simulink model "s_b4a4x256f"  (R2016b)
settings: Solver=VariableStepDiscrete  StartTime=0.0  StopTime=1  RelTol=1e-3
undefined symbols (not defined in the file): fft_stages, n_bits_ants, n_bits_xengs
libraries: xbsIndex_r4 x19303, casper_library_misc x166, casper_library_scopes x10, xbsReplacements_r4 x9, casper_library_delays x8, xps_library x3
(part 47 of 165)

== system s_b4a4x256f/sys0/31->32/conv8 ==
  note: (ones_bit & 1) -> round-to-even
      | (ones_bit ^ 1) -> round-to-odd
      | (sign_bit & 1)-> round-to-zero
      | (sign_bit ^ 1) -> round-to-inf
      | (X ~| 1) -> round half down
      | (X | 1) -> round half up
  in : Inport
  Concat : xbsIndex_r4/Concat  num_inputs=2  dbl_ovrd=off  block_type=concat
      settings: block_version=10.1.3
  Constant : xbsIndex_r4/Constant  const=1  gui_display_data_type=Fixed-point  arith_type=Unsigned  n_bits=1  bin_pt=0  preci_type=Single  exp_width=8  frac_width=24  explicit_period=off  period=1  equ=P=C  opselect=C  inp2=PCIN>>17  opr=+  inp1=P  carry=CIN  dbl_ovrd=off  block_type=constant
  Reinterpret : xbsIndex_r4/Reinterpret  force_arith_type=on  arith_type=Unsigned  force_bin_pt=on  bin_pt=0  block_type=reinterpret
      settings: infoedit="Changes signal type without altering the binary representation.   You can changed the signal between signed and unsigned, and relocate the binary point.<P><P>Hardware notes: In hardware this block costs nothing.<P><P>Example:  Suppose the input is 6 bits wide, signed, with 2 fractional bits, and the output is forced to unsigned with 0 fractional bits.  Then an input of -2.0 (1110.00 in binary 2's complement) becomes an output of 56 (111000 in binary)."  block_version=10.1.3
  adder : xbsIndex_r4/AddSub  mode=Addition  use_carryin=off  use_carryout=off  en=off  latency=0  precision=User Defined  arith_type="Signed  (2's comp)"  n_bits=32  bin_pt=0  quantization=Truncate  overflow=Wrap  use_behavioral_HDL=off  hw_selection=Fabric  pipelined=on  use_rpm=on  dbl_ovrd=off  block_type=addsub
      settings: xl_area=[0, 0, 0, 0, 0, 0, 0]  block_version=10.1.3
  almost_half : xbsIndex_r4/Constant  const=0  gui_display_data_type=Fixed-point  arith_type=Unsigned  n_bits=1  bin_pt=0  preci_type=Single  exp_width=8  frac_width=24  explicit_period=off  period=1  equ=P=C  opselect=C  inp2=PCIN>>17  opr=+  inp1=P  carry=CIN  dbl_ovrd=off  block_type=constant
  bit : xbsIndex_r4/Slice  nbits=1  boolean_output=off  mode=Lower Bit Location + Width  bit1=0  base1=MSB of Input  bit0=0  base0=LSB of Input  dbl_ovrd=off  block_type=slice
      settings: infoedit="Extracts a given range of bits from each input sample and presents it at the output.  The output type is ordinarily unsigned with binary point at zero, but can be Boolean when the slice is one bit wide.<P><P>Hardware notes: In hardware this block costs nothing."  block_version=10.1.3
  force1 : xbsIndex_r4/Reinterpret  force_arith_type=on  arith_type="Signed  (2's comp)"  force_bin_pt=on  bin_pt=1  block_type=reinterpret
      settings: infoedit="Changes signal type without altering the binary representation.   You can changed the signal between signed and unsigned, and relocate the binary point.<P><P>Hardware notes: In hardware this block costs nothing.<P><P>Example:  Suppose the input is 6 bits wide, signed, with 2 fractional bits, and the output is forced to unsigned with 0 fractional bits.  Then an input of -2.0 (1110.00 in binary 2's complement) becomes an output of 56 (111000 in binary)."  block_version=10.1.3
  force2 : xbsIndex_r4/Reinterpret  force_arith_type=off  arith_type="Signed  (2's comp)"  force_bin_pt=on  bin_pt=1  block_type=reinterpret
      settings: infoedit="Changes signal type without altering the binary representation.   You can changed the signal between signed and unsigned, and relocate the binary point.<P><P>Hardware notes: In hardware this block costs nothing.<P><P>Example:  Suppose the input is 6 bits wide, signed, with 2 fractional bits, and the output is forced to unsigned with 0 fractional bits.  Then an input of -2.0 (1110.00 in binary 2's complement) becomes an output of 56 (111000 in binary)."  block_version=10.1.3
  tweak_op : xbsIndex_r4/Logical  logical_function=NOR  inputs=2  en=off  latency=0  precision=Full  arith_type=Unsigned  n_bits=8  bin_pt=2  align_bp=on  dbl_ovrd=off  block_type=logical
      settings: xl_area=[0, 0, 0, 0, 0, 0, 0]
  out : Outport
  wires:
  tweak_op/1 -> Concat/2
  Constant/1 -> tweak_op/2
  bit/1 -> tweak_op/1
  almost_half/1 -> force2/1
  in/1 -> Reinterpret/1, bit/1
  Concat/1 -> force1/1
  Reinterpret/1 -> Concat/1
  force1/1 -> adder/1
  force2/1 -> adder/2
  adder/1 -> out/1

== system s_b4a4x256f/sys0/31->32/debus ==
  bus_in : Inport
  reinterpret{1..8} (8 alike) : xbsIndex_r4/Reinterpret  force_arith_type=on  arith_type="Signed  (2's comp)"  force_bin_pt=on  bin_pt=0  block_type=reinterpret
  slice1 : xbsIndex_r4/Slice  nbits=31  boolean_output=off  mode=Upper Bit Location + Width  bit1=-217  base1=MSB of Input  bit0=0  base0=LSB of Input  dbl_ovrd=off  block_type=slice
  slice2 : xbsIndex_r4/Slice  nbits=31  boolean_output=off  mode=Upper Bit Location + Width  bit1=-186  base1=MSB of Input  bit0=0  base0=LSB of Input  dbl_ovrd=off  block_type=slice
  slice3 : xbsIndex_r4/Slice  nbits=31  boolean_output=off  mode=Upper Bit Location + Width  bit1=-155  base1=MSB of Input  bit0=0  base0=LSB of Input  dbl_ovrd=off  block_type=slice
  slice4 : xbsIndex_r4/Slice  nbits=31  boolean_output=off  mode=Upper Bit Location + Width  bit1=-124  base1=MSB of Input  bit0=0  base0=LSB of Input  dbl_ovrd=off  block_type=slice
  slice5 : xbsIndex_r4/Slice  nbits=31  boolean_output=off  mode=Upper Bit Location + Width  bit1=-93  base1=MSB of Input  bit0=0  base0=LSB of Input  dbl_ovrd=off  block_type=slice
  slice6 : xbsIndex_r4/Slice  nbits=31  boolean_output=off  mode=Upper Bit Location + Width  bit1=-62  base1=MSB of Input  bit0=0  base0=LSB of Input  dbl_ovrd=off  block_type=slice
  slice7 : xbsIndex_r4/Slice  nbits=31  boolean_output=off  mode=Upper Bit Location + Width  bit1=-31  base1=MSB of Input  bit0=0  base0=LSB of Input  dbl_ovrd=off  block_type=slice
  slice8 : xbsIndex_r4/Slice  nbits=31  boolean_output=off  mode=Upper Bit Location + Width  bit1=0  base1=MSB of Input  bit0=0  base0=LSB of Input  dbl_ovrd=off  block_type=slice
  msb_out8 : Outport
  out7 : Outport  Port=2
  out6 : Outport  Port=3
  out5 : Outport  Port=4
  out4 : Outport  Port=5
  out3 : Outport  Port=6
  out2 : Outport  Port=7
  lsb_out1 : Outport  Port=8
  wires:
  bus_in/1 -> slice8/1, slice7/1, slice6/1, slice5/1, slice4/1, slice3/1, slice2/1, slice1/1
  slice8/1 -> reinterpret8/1
  reinterpret8/1 -> msb_out8/1
  slice7/1 -> reinterpret7/1
  reinterpret7/1 -> out7/1
  slice6/1 -> reinterpret6/1
  reinterpret6/1 -> out6/1
  slice5/1 -> reinterpret5/1
  reinterpret5/1 -> out5/1
  slice4/1 -> reinterpret4/1
  reinterpret4/1 -> out4/1
  slice3/1 -> reinterpret3/1
  reinterpret3/1 -> out3/1
  slice2/1 -> reinterpret2/1
  reinterpret2/1 -> out2/1
  slice1/1 -> reinterpret1/1
  reinterpret1/1 -> lsb_out1/1

== system s_b4a4x256f/sys0/beng_tvg/Delay10 ==
  d : Inport
  q : Outport
  wires:
  d/1 -> q/1

== system s_b4a4x256f/sys0/beng_tvg/Delay11 ==
  d : Inport
  q : Outport
  wires:
  d/1 -> q/1

== system s_b4a4x256f/sys0/beng_tvg/Delay52 ==
  d : Inport
  Register0 : xbsIndex_r4/Register  init=0  rst=off  en=off  dbl_ovrd=off  block_type=register
      settings: block_version=11.4
  q : Outport
  wires:
  Register0/1 -> q/1
  d/1 -> Register0/1

== system s_b4a4x256f/sys0/beng_tvg/Delay9 ==
  d : Inport
  q : Outport
  wires:
  d/1 -> q/1

== system s_b4a4x256f/sys0/bf/fbf ==
  note: beam filtering
  note: requanitse
  note: accumulate
  note: combine data from different antennas into beams
  note: beam steering
  note: antenna beam weights
  note: split polarisations and
      | duplicate for multiple beams
  note: TODO
  note: control interface
  note: TODO
  di : Inport
  deni : Inport  Port=2
  badi : Inport  Port=3
  timei : Inport  Port=4
  misci : Inport  Port=5
  ld_antenna : Inport  Port=6
  ld_stream : Inport  Port=7
  Assert1 : xbsIndex_r4/Assert  assert_type=on  type_source=Explicitly  gui_display_data_type=Boolean  arith_type=Boolean  n_bits=16  bin_pt=14  preci_type=Single  exp_width=8  frac_width=24  assert_rate=off  rate_source=Explicitly  period=1  output_port=on  block_type=assert
  Assert2 : xbsIndex_r4/Assert  assert_type=on  type_source=Explicitly  gui_display_data_type=Boolean  arith_type=Boolean  n_bits=16  bin_pt=14  preci_type=Single  exp_width=8  frac_width=24  assert_rate=off  rate_source=Explicitly  period=1  output_port=on  block_type=assert
  Assert3 : xbsIndex_r4/Assert  assert_type=on  type_source=Explicitly  gui_display_data_type=Fixed-point  arith_type=Unsigned  n_bits=n_bits_in*2*2^polarisation_bits  bin_pt=0  preci_type=Single  exp_width=8  frac_width=24  assert_rate=off  rate_source=Explicitly  period=1  output_port=on  block_type=assert
  Assert4 : xbsIndex_r4/Assert  assert_type=on  type_source=Explicitly  gui_display_data_type=Fixed-point  arith_type=Unsigned  n_bits=timestamp_bits  bin_pt=0  preci_type=Single  exp_width=8  frac_width=24  assert_rate=off  rate_source=Explicitly  period=1  output_port=on  block_type=assert
  Assert6 : xbsIndex_r4/Assert  assert_type=on  type_source=Explicitly  gui_display_data_type=Fixed-point  arith_type=Unsigned  n_bits=ant_bits  bin_pt=0  preci_type=Single  exp_width=8  frac_width=24  assert_rate=off  rate_source=Explicitly  period=1  output_port=on  block_type=assert
  Assert7 : xbsIndex_r4/Assert  assert_type=on  type_source=Explicitly  gui_display_data_type=Fixed-point  arith_type=Unsigned  n_bits=polarisation_bits+beam_bits  bin_pt=0  preci_type=Single  exp_width=8  frac_width=24  assert_rate=off  rate_source=Explicitly  period=1  output_port=on  block_type=assert
  Concat : xbsIndex_r4/Concat  num_inputs=2  dbl_ovrd=off  block_type=concat
  Concat1 : xbsIndex_r4/Concat  num_inputs=3  dbl_ovrd=off  block_type=concat
  Concat2 : xbsIndex_r4/Concat  num_inputs=2  dbl_ovrd=off  block_type=concat
  Concat3 : xbsIndex_r4/Concat  num_inputs=2  dbl_ovrd=off  block_type=concat
  Constant : xbsIndex_r4/Constant  const=0  gui_display_data_type=Boolean  arith_type=Boolean  n_bits=16  bin_pt=14  preci_type=Single  exp_width=8  frac_width=24  explicit_period=on  period=1  equ=P=C  opselect=C  inp2=PCIN>>17  opr=+  inp1=P  carry=CIN  dbl_ovrd=off  block_type=constant
  Constant1 : xbsIndex_r4/Constant  const=0  gui_display_data_type=Fixed-point  arith_type=Unsigned  n_bits=1  bin_pt=0  preci_type=Single  exp_width=8  frac_width=24  explicit_period=on  period=1  equ=P=C  opselect=C  inp2=PCIN>>17  opr=+  inp1=P  carry=CIN  dbl_ovrd=off  block_type=constant
  Delay : xbsIndex_r4/Delay  rst=off  infoeditControl=Selection of Reset will increase slice count due to use of real FFs and instead of SRLs  en=on  latency=1  reg_retiming=off  dbl_ovrd=off  block_type=delay
      settings: infoedit=Hardware notes: A delay line is a chain, each link of which is an SRL16 or SRL32 followed by a flip-flop.
  Delay1 : xbsIndex_r4/Delay  rst=off  infoeditControl=Selection of Reset will increase slice count due to use of real FFs and instead of SRLs  en=off  latency=1  reg_retiming=on  dbl_ovrd=off  block_type=delay
  Delay13 : xbsIndex_r4/Delay  rst=off  infoeditControl=Selection of Reset will increase slice count due to use of real FFs and instead of SRLs  en=off  latency=1  reg_retiming=on  dbl_ovrd=off  block_type=delay
  Delay2 : xbsIndex_r4/Delay  rst=off  infoeditControl=Selection of Reset will increase slice count due to use of real FFs and instead of SRLs  en=off  latency=1  reg_retiming=on  dbl_ovrd=off  block_type=delay
  Delay{4..6,8..9} (5 alike) : xbsIndex_r4/Delay  rst=off  infoeditControl=Selection of Reset will increase slice count due to use of real FFs and instead of SRLs  en=off  latency=1  reg_retiming=off  dbl_ovrd=off  block_type=delay
      settings: infoedit=Hardware notes: A delay line is a chain, each link of which is an SRL16 or SRL32 followed by a flip-flop.
  Delay7 : xbsIndex_r4/Delay  rst=off  infoeditControl=Selection of Reset will increase slice count due to use of real FFs and instead of SRLs  en=on  latency=1  reg_retiming=off  dbl_ovrd=off  block_type=delay
      settings: infoedit=Hardware notes: A delay line is a chain, each link of which is an SRL16 or SRL32 followed by a flip-flop.
  Gateway Out{,1..6,10..16,18..24} (21 alike) : xbsIndex_r4/Gateway Out  inherit_from_input=off  hdl_port=off  rows=1  columns=1  UseAsDAC=off  DACChannel='1'  interface=None  automatic_assignment=on  address_offset=hex2dec('00')  intf_name=''  intf_description=''  timing_constraint=None  locs_specified=off  LOCs={}  io_standard={}  block_type=gatewayout
      settings: infoedit="Gateway out block.  Converts Xilinx fixed point inputs into ouputs of type Simulink integer, double, or fixed point.<br><br>Hardware notes:  In hardware these blocks become top level output ports or are discarded, depending on how they are configured."  block_version=11.4
  Reinterpret : xbsIndex_r4/Reinterpret  force_arith_type=on  arith_type="Signed  (2's comp)"  force_bin_pt=on  bin_pt=bin_pt_in+bin_pt_norm  block_type=reinterpret
  Reinterpret1 : xbsIndex_r4/Reinterpret  force_arith_type=on  arith_type="Signed  (2's comp)"  force_bin_pt=on  bin_pt=bin_pt_in+bin_pt_norm  block_type=reinterpret
  Reinterpret11 : xbsIndex_r4/Reinterpret  force_arith_type=on  arith_type=Unsigned  force_bin_pt=on  bin_pt=0  block_type=reinterpret
  Reinterpret12 : xbsIndex_r4/Reinterpret  force_arith_type=on  arith_type=Unsigned  force_bin_pt=on  bin_pt=0  block_type=reinterpret
  Reinterpret2 : xbsIndex_r4/Reinterpret  force_arith_type=on  arith_type="Signed  (2's comp)"  force_bin_pt=on  bin_pt=bin_pt_out  block_type=reinterpret
  Reinterpret3 : xbsIndex_r4/Reinterpret  force_arith_type=on  arith_type="Signed  (2's comp)"  force_bin_pt=on  bin_pt=bin_pt_out  block_type=reinterpret
  Reinterpret5 : xbsIndex_r4/Reinterpret  force_arith_type=on  arith_type="Signed  (2's comp)"  force_bin_pt=on  bin_pt=bin_pt_norm  block_type=reinterpret
  Reinterpret6 : xbsIndex_r4/Reinterpret  force_arith_type=on  arith_type=Unsigned  force_bin_pt=on  bin_pt=0  block_type=reinterpret
  Scope : Scope  NumInputPorts=5
  Scope1 : Scope  NumInputPorts=4
  Scope3 : Scope  NumInputPorts=6
  Scope4 : Scope  NumInputPorts=6
  Slice : xbsIndex_r4/Slice  nbits=n_bits_combine  boolean_output=off  mode=Lower Bit Location + Width  bit1=0  base1=MSB of Input  bit0=0  base0=LSB of Input  dbl_ovrd=off  block_type=slice
  Slice1 : xbsIndex_r4/Slice  nbits=n_bits_combine  boolean_output=off  mode=Upper Bit Location + Width  bit1=0  base1=MSB of Input  bit0=n_bits_combine  base0=LSB of Input  dbl_ovrd=off  block_type=slice
  Slice2 : xbsIndex_r4/Slice  nbits=n_bits_out  boolean_output=off  mode=Lower Bit Location + Width  bit1=0  base1=MSB of Input  bit0=0  base0=LSB of Input  dbl_ovrd=off  block_type=slice
  Slice3 : xbsIndex_r4/Slice  nbits=n_bits_out  boolean_output=off  mode=Lower Bit Location + Width  bit1=0  base1=MSB of Input  bit0=n_bits_out  base0=LSB of Input  dbl_ovrd=off  block_type=slice
  Slice6 : xbsIndex_r4/Slice  nbits=timestamp_bits  boolean_output=off  mode=Upper Bit Location + Width  bit1=-1  base1=MSB of Input  bit0=n_bits_combine  base0=LSB of Input  dbl_ovrd=off  block_type=slice
  Slice9 : xbsIndex_r4/Slice  nbits=n_bits_out  boolean_output=on  mode=Upper Bit Location + Width  bit1=0  base1=MSB of Input  bit0=0  base0=LSB of Input  dbl_ovrd=off  block_type=slice
  apply_beam_weights : Subsystem  mask{vec_bits=ant_bits, stream_bits=polarisation_bits+beam_bits, stack_bits=stack_bits, type_in=1, n_bits_in=n_bits_in, bin_pt_in=bin_pt_in, complex_in=on, type_coeff=1, n_bits_coeff=n_bits_norm, bin_pt_coeff=bin_pt_norm, complex_coeff=off, mult_latency=mult_latency, conv_latency=0, n_bits_out=n_bits_in+n_bits_norm+1, bin_pt_out=bin_pt_in+bin_pt_norm, type_out=1, quantization=0, overflow=0, init_val=1}
      mask prompts: vec_bits "vector length (2^?)"; stream_bits "streams (2^?)"; stack_bits "stack factor (2^?)"; type_in "input type (Unsigned=0, Signed=1)"; n_bits_in "bit width in"; bin_pt_in "binary point in"; complex_in "complex input"; type_coeff "coefficient type (Unsigned=0, Signed=1)"; n_bits_coeff "coefficient bit width"; bin_pt_coeff "coefficient binary point"; complex_coeff "complex coefficients"; mult_latency "multiplier latency"; conv_latency "convert latency"; n_bits_out "output bit width"; bin_pt_out "output binary point"; type_out "output type (Unsigned=0, Signed=1)"; quantization "quantization strategy (Truncate=0, Round  (unbiased: +/- Inf)=1)"; overflow "overflow strategy (Wrap=0, Saturate=1, Flag as error=2)"; init_val "initial value"
      mask init:
      | if strcmp(complex_in, 'on'),
      |     set_param([gcb, '/munge_in'], ...
      |         'divisions', '2^stream_bits', ...
      |         'div_size', 'repmat(n_bits_in*2, 1, 2^stream_bits)', ...
      |         'order', 'max(0,2^stream_bits-1):-1:0');
      |     set_param([gcb, '/munge_out'], ...
      |         'divisions', '2^stream_bits', ...
      |         'div_size', 'repmat(n_bits_out*2, 1, 2^stream_bits)', ...
      |         'order', 'max(0,2^stream_bits-1):-1:0');    
      | else
      |     set_param([gcb, '/munge_in'], ...
      |         'divisions', '2^stream_bits', ...
      |         'div_size', 'repmat(n_bits_in, 1, 2^stream_bits)', ...
      |         'order', 'max(0,2^stream_bits-1):-1:0');
      |     set_param([gcb, '/munge_out'], ...
      |         'divisions', '2^stream_bits', ...
      |         'div_size', 'repmat(n_bits_out, 1, 2^stream_bits)', ...
      |         'order', 'max(0,2^stream_bits-1):-1:0');    
      | end
      | 
      | set_param([gcb,'/bus_mult'], ...
      |     'n_bits_b', 'repmat(n_bits_coeff, 1, 2^stream_bits)', ...
      |     'bin_pt_b', 'bin_pt_coeff', ...
      |     'type_b', 'type_coeff', 'cmplx_b', complex_coeff, ...
      |     'n_bits_a', 'repmat(n_bits_in, 1, 2^stream_bits)', ...
      |     'bin_pt_a', 'bin_pt_in', ... 
      |     'type_a', 'type_in', 'cmplx_a', complex_in, ...
      |     'n_bits_out', 'n_bits_coeff+n_bits_in+1', ...
      |     'bin_pt_out', 'bin_pt_coeff+bin_pt_in', ...
      |     'type_out', 'type_out', ...
      |     'quantization', '0', 'overflow', '0', ... 
      |     'mult_latency', 'mult_latency');
      | 
      | set_param([gcb,'/bus_convert'], ...
      |     'n_bits_in', 'repmat(n_bits_coeff+n_bits_in+1, 1, 2^stream_bits)', ...
      |     'bin_pt_in', 'bin_pt_coeff+bin_pt_in', ...
      |     'cmplx', complex_in, ...
      |     'n_bits_out', 'n_bits_out', ...
      |     'bin_pt_out', 'bin_pt_out', ...
      |     'quantization', 'quantization', 'overflow', 'overflow', ... 
      |     'latency', 'conv_latency')
      | 
      | if strcmp(complex_coeff, 'on'),
      |     set_param([gcb,'/dinb'], ...
      |         'n_bits', 'n_bits_coeff*2*2^stream_bits');
      |     set_param([gcb,'/coeffs'], ...
      |         'depth', '2^(vec_bits+stream_bits)', ...
      |         'initVector', 'repmat(real(init_val)*2^(bin_pt_coeff+n_bits_coeff)+imag(init_val)*2^(bin_pt_coeff),1,2^(vec_bits+stream_bits))');
      | else
      |     set_param([gcb,'/dinb'], ...
      |         'n_bits', 'n_bits_coeff*2^stream_bits');
      |     set_param([gcb,'/coeffs'], ...
      |         'depth', '2^(vec_bits+stream_bits)', ...
      |         'initVector', 'repmat(real(init_val)*2^(bin_pt_coeff),1,2^(vec_bits+stream_bits))');
      | end
  bad_slc : xbsIndex_r4/Slice  nbits=1  boolean_output=on  mode=Upper Bit Location + Width  bit1=0  base1=MSB of Input  bit0=0  base0=LSB of Input  dbl_ovrd=off  block_type=slice
  bus_expand : Subsystem  AncestorBlock=casper_library_flow_control/bus_expand  mask(bus_expand){mode=divisions of equal size, outputNum=4, outputWidth=n_bits_in, outputBinaryPt=bin_pt_in, outputArithmeticType=1, show_format=off, outputToWorkspace=off, variablePrefix=out, outputToModelAsWell=on}
      mask prompts: outputNum "Number of outputs:"; outputWidth "Output width:"; outputBinaryPt "Output binary point position:"; outputArithmeticType "Output arithmetic type (ufix=0, fix=1, bool=2):"; show_format "Print format string?"; outputToWorkspace "Output to workspace?"; variablePrefix "Variable name prefix:"; outputToModelAsWell "Output to model as well?"
      mask help:
      | Expands a 'bus' made using a bus_create or Xilinx
      | concat block.
      | The input will be divided into the specified number
      | of outputs with the specified arithmetic types.
      | Divisions are made from most significant bit.
      mask init: same as s_b4a4x256f/bus_expand
      settings: AttributesFormatString=4 outputs
      mask TypeOptions mode: divisions of equal size | divisions of arbitrary size
      mask Callback mode: bus_expand_callback();
      mask Callback outputWidth: bus_expand_callback();
      mask Callback outputToWorkspace: bus_expand_callback();
  bus_expand1 : Subsystem  AncestorBlock=casper_library_flow_control/bus_expand  mask(bus_expand){mode=divisions of equal size, outputNum=4, outputWidth=n_bits_in+n_bits_norm+1, outputBinaryPt=bin_pt_in+bin_pt_norm, outputArithmeticType=1, show_format=off, outputToWorkspace=off, variablePrefix=out, outputToModelAsWell=on}
      mask prompts: outputNum "Number of outputs:"; outputWidth "Output width:"; outputBinaryPt "Output binary point position:"; outputArithmeticType "Output arithmetic type (ufix=0, fix=1, bool=2):"; show_format "Print format string?"; outputToWorkspace "Output to workspace?"; variablePrefix "Variable name prefix:"; outputToModelAsWell "Output to model as well?"
      mask help:
      | Expands a 'bus' made using a bus_create or Xilinx
      | concat block.
      | The input will be divided into the specified number
      | of outputs with the specified arithmetic types.
      | Divisions are made from most significant bit.
      mask init: same as s_b4a4x256f/bus_expand
      settings: AttributesFormatString=4 outputs
      mask TypeOptions mode: divisions of equal size | divisions of arbitrary size
      mask Callback mode: bus_expand_callback();
      mask Callback outputWidth: bus_expand_callback();
      mask Callback outputToWorkspace: bus_expand_callback();
  combine : Subsystem  mask{freq_bits=freq_bits-beng_bits, ant_bits=ant_bits, stack_bits=stack_bits, stream_bits=beam_bits+polarisation_bits, n_bits_in=n_bits_in+n_bits_norm+1, bin_pt_in=bin_pt_in+bin_pt_norm, timestamp_bits=timestamp_bits, n_bits_accum=n_bits_combine, bram_latency=bram_latency, add_latency=add_latency}
      mask prompts: freq_bits "frequencies (2^?)"; ant_bits "antennas (2^?)"; stack_bits "stacking factor (2^?)"; stream_bits "input streams (2^?)"; n_bits_in "data bits in"; bin_pt_in "binary point in"; timestamp_bits "timestamp bits"; n_bits_accum "accumulator bits"; bram_latency "bram latency"; add_latency "add latency"
  duplicate : Subsystem  mask{ant_bits=ant_bits, freq_bits=freq_bits-beng_bits, stack_bits=stack_bits, beam_bits=beam_bits, polarisation_bits=polarisation_bits, n_bits_in=n_bits_in}
      mask prompts: ant_bits "antennas (2^?)"; freq_bits "frequencies (2^?)"; stack_bits "stacking factor (2^?)"; beam_bits "beams (2^?)"; polarisation_bits "polarisations (2^?)"; n_bits_in "data bits in"
      mask init:
      | set_param([gcb,'/beam_replicate'], ...
      |     'replication', '2^beam_bits');
      | set_param([gcb,'/pol_replicate'], ...
      |     'replication', '2^polarisation_bits');
  ld_freq5 : xbsIndex_r4/Slice  nbits=1  boolean_output=off  mode=Two Bit Locations  bit1=-(timestamp_bits+1)  base1=MSB of Input  bit0=0  base0=LSB of Input  dbl_ovrd=off  block_type=slice
  misco_slc : xbsIndex_r4/Slice  nbits=1  boolean_output=off  mode=Two Bit Locations  bit1=-timestamp_bits  base1=MSB of Input  bit0=0  base0=LSB of Input  dbl_ovrd=off  block_type=slice
  pipeline1 : Subsystem  AncestorBlock=casper_library_delays/pipeline  mask(pipeline){latency=2}
      mask help:
      | An explicitly laid-out delay line to avoid mapping to SRL16s
      | for use in pipelining to help achieve timing closure.
      mask init:
      | pipeline_init(gcb,'latency',latency);
      settings: AttributesFormatString=Latency = %<latency>
      mask Display:
      | port_label('input', 1, 'd');
      | port_label('output', 1, 'q');
      | disp(['Z^-', num2str(latency)]);
  pipeline10 : Subsystem  AncestorBlock=casper_library_delays/pipeline  mask(pipeline){latency=2}
      mask help:
      | An explicitly laid-out delay line to avoid mapping to SRL16s
      | for use in pipelining to help achieve timing closure.
      mask init:
      | pipeline_init(gcb,'latency',latency);
      settings: AttributesFormatString=Latency = %<latency>
      mask Display:
      | port_label('input', 1, 'd');
      | port_label('output', 1, 'q');
      | disp(['Z^-', num2str(latency)]);
  pipeline11 : Subsystem  AncestorBlock=casper_library_delays/pipeline  mask(pipeline){latency=2}
      mask help:
      | An explicitly laid-out delay line to avoid mapping to SRL16s
      | for use in pipelining to help achieve timing closure.
      mask init:
      | pipeline_init(gcb,'latency',latency);
      settings: AttributesFormatString=Latency = %<latency>
      mask Display:
      | port_label('input', 1, 'd');
      | port_label('output', 1, 'q');
      | disp(['Z^-', num2str(latency)]);
  pipeline12 : Subsystem  AncestorBlock=casper_library_delays/pipeline  mask(pipeline){latency=2}
      mask help:
      | An explicitly laid-out delay line to avoid mapping to SRL16s
      | for use in pipelining to help achieve timing closure.
      mask init:
      | pipeline_init(gcb,'latency',latency);
      settings: AttributesFormatString=Latency = %<latency>
      mask Display:
      | port_label('input', 1, 'd');
      | port_label('output', 1, 'q');
      | disp(['Z^-', num2str(latency)]);
  pipeline13 : Subsystem  AncestorBlock=casper_library_delays/pipeline  mask(pipeline){latency=2}
      mask help:
      | An explicitly laid-out delay line to avoid mapping to SRL16s
      | for use in pipelining to help achieve timing closure.
      mask init:
      | pipeline_init(gcb,'latency',latency);
      settings: AttributesFormatString=Latency = %<latency>
      mask Display:
      | port_label('input', 1, 'd');
      | port_label('output', 1, 'q');
      | disp(['Z^-', num2str(latency)]);
  pipeline14 : Subsystem  AncestorBlock=casper_library_delays/pipeline  mask(pipeline){latency=2}
      mask help:
      | An explicitly laid-out delay line to avoid mapping to SRL16s
      | for use in pipelining to help achieve timing closure.
      mask init:
      | pipeline_init(gcb,'latency',latency);
      settings: AttributesFormatString=Latency = %<latency>
      mask Display:
      | port_label('input', 1, 'd');
      | port_label('output', 1, 'q');
      | disp(['Z^-', num2str(latency)]);
  pipeline15 : Subsystem  AncestorBlock=casper_library_delays/pipeline  mask(pipeline){latency=2}
      mask help:
      | An explicitly laid-out delay line to avoid mapping to SRL16s
      | for use in pipelining to help achieve timing closure.
      mask init:
      | pipeline_init(gcb,'latency',latency);
      settings: AttributesFormatString=Latency = %<latency>
      mask Display:
      | port_label('input', 1, 'd');
      | port_label('output', 1, 'q');
      | disp(['Z^-', num2str(latency)]);
  pipeline16 : Subsystem  AncestorBlock=casper_library_delays/pipeline  mask(pipeline){latency=2}
      mask help:
      | An explicitly laid-out delay line to avoid mapping to SRL16s
      | for use in pipelining to help achieve timing closure.
      mask init:
      | pipeline_init(gcb,'latency',latency);
      settings: AttributesFormatString=Latency = %<latency>
      mask Display:
      | port_label('input', 1, 'd');
      | port_label('output', 1, 'q');
      | disp(['Z^-', num2str(latency)]);
  pipeline2 : Subsystem  AncestorBlock=casper_library_delays/pipeline  mask(pipeline){latency=2}
      mask help:
      | An explicitly laid-out delay line to avoid mapping to SRL16s
      | for use in pipelining to help achieve timing closure.
      mask init:
      | pipeline_init(gcb,'latency',latency);
      settings: AttributesFormatString=Latency = %<latency>
      mask Display:
      | port_label('input', 1, 'd');
      | port_label('output', 1, 'q');
      | disp(['Z^-', num2str(latency)]);
  pipeline3 : Subsystem  AncestorBlock=casper_library_delays/pipeline  mask(pipeline){latency=2}
      mask help:
      | An explicitly laid-out delay line to avoid mapping to SRL16s
      | for use in pipelining to help achieve timing closure.
      mask init:
      | pipeline_init(gcb,'latency',latency);
      settings: AttributesFormatString=Latency = %<latency>
      mask Display:
      | port_label('input', 1, 'd');
      | port_label('output', 1, 'q');
      | disp(['Z^-', num2str(latency)]);
  pipeline8 : Subsystem  AncestorBlock=casper_library_delays/pipeline  mask(pipeline){latency=2}
      mask help:
      | An explicitly laid-out delay line to avoid mapping to SRL16s
      | for use in pipelining to help achieve timing closure.
      mask init:
      | pipeline_init(gcb,'latency',latency);
      settings: AttributesFormatString=Latency = %<latency>
      mask Display:
      | port_label('input', 1, 'd');
      | port_label('output', 1, 'q');
      | disp(['Z^-', num2str(latency)]);
  pipeline9 : Subsystem  AncestorBlock=casper_library_delays/pipeline  mask(pipeline){latency=2}
      mask help:
      | An explicitly laid-out delay line to avoid mapping to SRL16s
      | for use in pipelining to help achieve timing closure.
      mask init:
      | pipeline_init(gcb,'latency',latency);
      settings: AttributesFormatString=Latency = %<latency>
      mask Display:
      | port_label('input', 1, 'd');
      | port_label('output', 1, 'q');
      | disp(['Z^-', num2str(latency)]);
  requantise : Subsystem  mask{vec_bits=freq_bits-beng_bits, stream_bits=polarisation_bits+beam_bits, stack_bits=stack_bits, type_in=1, n_bits_in=n_bits_combine, bin_pt_in=bin_pt_in+bin_pt_norm, complex_in=on, type_coeff=1, n_bits_coeff=n_bits_requant, bin_pt_coeff=bin_pt_requant, complex_coeff=off, mult_latency=mult_latency, conv_latency=conv_latency, n_bits_out=n_bits_out, bin_pt_out=bin_pt_out, type_out=1, quantization=1, overflow=1, init_val=1}
      mask prompts: vec_bits "vector length (2^?)"; stream_bits "streams (2^?)"; stack_bits "stack factor (2^?)"; type_in "input type (Unsigned=0, Signed=1)"; n_bits_in "bit width in"; bin_pt_in "binary point in"; complex_in "complex input"; type_coeff "coefficient type (Unsigned=0, Signed=1)"; n_bits_coeff "coefficient bit width"; bin_pt_coeff "coefficient binary point"; complex_coeff "complex coefficients"; mult_latency "multiplier latency"; conv_latency "convert latency"; n_bits_out "output bit width"; bin_pt_out "output binary point"; type_out "output type (Unsigned=0, Signed=1)"; quantization "quantization strategy (Truncate=0, Round  (unbiased: +/- Inf)=1)"; overflow "overflow strategy (Wrap=0, Saturate=1, Flag as error=2)"; init_val "initial value"
      mask init:
      | % if strcmp(complex_in, 'on'),
      | %     set_param([gcb, '/munge_in'], ...
      | %         'divisions', '2^stream_bits', ...
      | %         'div_size', 'repmat(n_bits_in*2, 1, 2^stream_bits)', ...
      | %         'order', 'max(0,2^stream_bits-1):-1:0');
      | %     set_param([gcb, '/munge_out'], ...
      | %         'divisions', '2^stream_bits', ...
      | %         'div_size', 'repmat(n_bits_out*2, 1, 2^stream_bits)', ...
      | %         'order', 'max(0,2^stream_bits-1):-1:0');    
      | % else
      | %     set_param([gcb, '/munge_in'], ...
      | %         'divisions', '2^stream_bits', ...
      | %         'div_size', 'repmat(n_bits_in, 1, 2^stream_bits)', ...
      | %         'order', 'max(0,2^stream_bits-1):-1:0');
      | %     set_param([gcb, '/munge_out'], ...
      | %         'divisions', '2^stream_bits', ...
      | %         'div_size', 'repmat(n_bits_out, 1, 2^stream_bits)', ...
      | %         'order', 'max(0,2^stream_bits-1):-1:0');    
      | % end
      | % 
      | % set_param([gcb,'/bus_mult'], ...
      | %     'n_bits_b', 'repmat(n_bits_coeff, 1, 2^stream_bits)', ...
      | %     'bin_pt_b', 'bin_pt_coeff', ...
      | %     'type_b', 'type_coeff', 'cmplx_b', complex_coeff, ...
      | %     'n_bits_a', 'repmat(n_bits_in, 1, 2^stream_bits)', ...
      | %     'bin_pt_a', 'bin_pt_in', ... 
      | %     'type_a', 'type_in', 'cmplx_a', complex_in, ...
      | %     'n_bits_out', 'n_bits_coeff+n_bits_in+1', ...
      | %     'bin_pt_out', 'bin_pt_coeff+bin_pt_in', ...
      | %     'type_out', 'type_out', ...
      | %     'quantization', '0', 'overflow', '0', ... 
      | %     'mult_latency', 'mult_latency');
      | % 
      | % set_param([gcb,'/bus_convert'], ...
      | %     'n_bits_in', 'repmat(n_bits_coeff+n_bits_in+1, 1, 2^stream_bits)', ...
      | %     'bin_pt_in', 'bin_pt_coeff+bin_pt_in', ...
      | %     'cmplx', complex_in, ...
      | %     'n_bits_out', 'n_bits_out', ...
      | %     'bin_pt_out', 'bin_pt_out', ...
      | %     'quantization', 'quantization', 'overflow', 'overflow', ... 
      | %     'latency', 'conv_latency')
      | % 
      | % if strcmp(complex_coeff, 'on'),
      | %     set_param([gcb,'/dinb'], ...
      | %         'n_bits', 'n_bits_coeff*2*2^stream_bits');
      | %     set_param([gcb,'/coeffs'], ...
      | %         'depth', '2^(vec_bits+stream_bits)', ...
      | %         'initVector', 'repmat(real(init_val)*2^(bin_pt_coeff+n_bits_coeff)+imag(init_val)*2^(bin_pt_coeff),1,2^(vec_bits+stream_bits))');
      | % else
      | %     set_param([gcb,'/dinb'], ...
      | %         'n_bits', 'n_bits_coeff*2^stream_bits');
      | %     set_param([gcb,'/coeffs'], ...
      | %         'depth', '2^(vec_bits+stream_bits)', ...
      | %         'initVector', 'repmat(real(init_val)*2^(bin_pt_coeff),1,2^(vec_bits+stream_bits))');
      | % end
  sync_gen : Subsystem
  time_slc : xbsIndex_r4/Slice  nbits=timestamp_bits  boolean_output=off  mode=Upper Bit Location + Width  bit1=-1  base1=MSB of Input  bit0=0  base0=LSB of Input  dbl_ovrd=off  block_type=slice
  timeo_slc : xbsIndex_r4/Slice  nbits=timestamp_bits  boolean_output=off  mode=Upper Bit Location + Width  bit1=0  base1=MSB of Input  bit0=0  base0=LSB of Input  dbl_ovrd=off  block_type=slice
  synco : Outport
  do : Outport  Port=2
  deno : Outport  Port=3
  timeo : Outport  Port=4
  misco : Outport  Port=5
  bw_value_out : Outport  Port=6
  wires:
  misci/1 -> sync_gen/5(misci)
  Assert4/1 -> sync_gen/4(timei)
  Assert2/1 -> sync_gen/3(badi)
  Assert3/1 -> sync_gen/2(di)
  Assert1/1 -> sync_gen/1(en)
  Assert7/1 -> [stream]
  ld_stream/1 -> Assert7/1
  Assert6/1 -> [antenna]
  ld_antenna/1 -> Assert6/1
  Gateway Out5/1 -> Scope1/4
  Gateway Out4/1 -> Scope1/3
  Gateway Out3/1 -> Scope1/2
  Gateway Out18/1 -> Scope1/1
  [requantise_synco] -> Delay9/1
  requantise/1(synco) -> [requantise_synco], synco/1
  [bw_val_out] -> Reinterpret5/1
  apply_beam_weights/4(misco) -> pipeline11/1(d), Slice6/1
  Gateway Out14/1 -> Scope3/6
  Gateway Out13/1 -> Scope3/5
  Gateway Out12/1 -> Scope3/4
  Gateway Out11/1 -> Scope3/3
  Gateway Out10/1 -> Scope3/2
  Gateway Out16/1 -> Scope3/1
  sync_gen/1(synco) -> [synco], duplicate/1(synci)
  Gateway Out6/1 -> Scope/5
  Gateway Out2/1 -> Scope/4
  Gateway Out1/1 -> Scope/3
  Gateway Out/1 -> Scope/2
  Gateway Out15/1 -> Scope/1
  [combine_sync] -> Delay4/1
  requantise/4(misco) -> misco_slc/1, timeo_slc/1
  requantise/3(eno) -> deno/1, [requantise_eno]
  requantise/2(dout) -> do/1, [requantise_dout]
  combine/1(synco) -> [combine_sync], pipeline15/1(d)
  apply_beam_weights/1(synco) -> pipeline8/1(d), [bw_synco]
  sync_gen/2(do) -> [do], duplicate/3(di)
  bus_expand/4(lsb_out1) -> Gateway Out13/1
  bus_expand/3(out2) -> Gateway Out12/1
  sync_gen/3(dvalid) -> [dvalid], duplicate/2(eni)
  bus_expand/2(out3) -> Gateway Out11/1
  bus_expand/1(msb_out4) -> Gateway Out10/1
  [combine_time] -> Delay6/1
  Concat3/1 -> pipeline3/1(d)
  combine/5(misco) -> Concat3/2
  combine/4(timeo) -> [combine_time], Concat3/1
  time_slc/1 -> combine/5(timei)
  Reinterpret3/1 -> Gateway Out4/1
  Reinterpret2/1 -> Gateway Out3/1
  [requantise_eno] -> Delay8/1, Slice9/1
  Slice2/1 -> Reinterpret3/1
  Slice3/1 -> Reinterpret2/1
  Reinterpret1/1 -> Gateway Out1/1
  Reinterpret/1 -> Gateway Out/1
  [combine_eno] -> Delay/2, Delay5/1
  Slice/1 -> Reinterpret1/1
  Slice1/1 -> Reinterpret/1
  apply_beam_weights/3(eno) -> pipeline10/1(d), [bw_eno]
  apply_beam_weights/2(dout) -> pipeline9/1(d), [bw_dout]
  combine/3(eno) -> [combine_eno], pipeline2/1(d)
  combine/2(sum) -> [combine_sum], pipeline1/1(d)
  [bf_valctrl_bw] -> Delay1/1
  Concat/1 -> Delay13/1
  timei/1 -> Assert4/1
  ld_freq5/1 -> combine/6(misci)
  bad_slc/1 -> combine/4(bad)
  badi/1 -> Assert2/1
  di/1 -> Assert3/1
  deni/1 -> Assert1/1
  [antenna] -> Concat/1
  [stream] -> Concat/2
  Delay2/1 -> apply_beam_weights/6(vali)
  Concat2/1 -> requantise/5(vali)
  [bf_value_bw] -> Reinterpret6/1
  pipeline15/1(q) -> requantise/1(synci)
  pipeline1/1(q) -> requantise/2(din)
  pipeline2/1(q) -> requantise/3(den)
  pipeline3/1(q) -> requantise/4(misci)
  pipeline8/1(q) -> combine/1(synci)
  pipeline9/1(q) -> combine/2(data)
  pipeline10/1(q) -> combine/3(den)
  pipeline11/1(q) -> time_slc/1, ld_freq5/1, bad_slc/1
  pipeline12/1(q) -> apply_beam_weights/1(synci)
  pipeline13/1(q) -> apply_beam_weights/2(din)
  pipeline14/1(q) -> apply_beam_weights/3(den)
  pipeline16/1(q) -> apply_beam_weights/4(misci)
  Slice6/1 -> [bfabw_time0]
  Concat1/1 -> pipeline16/1(d)
  sync_gen/4(bado) -> duplicate/4(badi)
  sync_gen/5(timeo) -> duplicate/5(timei)
  sync_gen/6(misco) -> duplicate/6(misci)
  duplicate/4(bado) -> Concat1/1
  duplicate/5(timeo) -> Concat1/2
  duplicate/6(misco) -> Concat1/3
  duplicate/3(eno) -> pipeline14/1(d)
  duplicate/2(do) -> pipeline13/1(d)
  duplicate/1(synco) -> pipeline12/1(d)
  Constant/1 -> duplicate/7(sim_ld)
  Constant1/1 -> duplicate/8(sim_type)
  Reinterpret12/1 -> Concat2/1
  Reinterpret11/1 -> Concat2/2
  [synco] -> Gateway Out16/1
  [do] -> bus_expand/1(bus_in)
  [dvalid] -> Gateway Out14/1
  Gateway Out23/1 -> Scope4/6
  Gateway Out22/1 -> Scope4/5
  Gateway Out21/1 -> Scope4/4
  Gateway Out20/1 -> Scope4/3
  Gateway Out19/1 -> Scope4/2
  Gateway Out24/1 -> Scope4/1
  bus_expand1/4(lsb_out1) -> Gateway Out22/1
  bus_expand1/3(out2) -> Gateway Out21/1
  bus_expand1/2(out3) -> Gateway Out20/1
  bus_expand1/1(msb_out4) -> Gateway Out19/1
  [bw_synco] -> Gateway Out24/1
  [bw_dout] -> bus_expand1/1(bus_in)
  [bw_eno] -> Gateway Out23/1
  [combine_sum] -> Delay/1
  Delay/1 -> Slice/1, Slice1/1
  Delay4/1 -> Gateway Out15/1
  Delay5/1 -> Gateway Out2/1
  Delay6/1 -> Gateway Out6/1
  Delay7/1 -> Slice2/1, Slice3/1
  [requantise_dout] -> Delay7/1
  Delay8/1 -> Gateway Out5/1
  Delay9/1 -> Gateway Out18/1
  Slice9/1 -> Delay7/2
  Reinterpret6/1 -> Delay2/1
  Delay13/1 -> apply_beam_weights/5(index)
  timeo_slc/1 -> timeo/1
  misco_slc/1 -> misco/1
  apply_beam_weights/5(valo) -> [bw_val_out]
  Reinterpret5/1 -> bw_value_out/1
  [bf0_gain] -> Reinterpret12/1
  [bf1_gain] -> Reinterpret11/1
  Delay1/1 -> apply_beam_weights/7(we)

== system s_b4a4x256f/sys0/bf_pack_out0/Subsystem3 ==
  rst : Inport
  in0 : Inport  Port=2
  in1 : Inport  Port=3
  Counter : xbsIndex_r4/Counter  cnt_type=Free Running  cnt_to=Inf  operation=Up  start_count=0  cnt_by_val=1  arith_type=Unsigned  n_bits=16  bin_pt=0  load_pin=off  rst=on  en=on  explicit_period=on  period=1  use_behavioral_HDL=on  implementation=Fabric  dbl_ovrd=off  block_type=counter
  Counter1 : xbsIndex_r4/Counter  cnt_type=Free Running  cnt_to=Inf  operation=Up  start_count=0  cnt_by_val=1  arith_type=Unsigned  n_bits=16  bin_pt=0  load_pin=off  rst=on  en=on  explicit_period=on  period=1  use_behavioral_HDL=on  implementation=Fabric  dbl_ovrd=off  block_type=counter
  edge_detect : casper_library_misc/edge_detect  edge=Rising  polarity=Active High  x_in=[0 0.08 0.08 0.16 0.16 0.24 0.24 0.32 0.32 0.4]  y_in="[-1 -1  1  1  1  1  1  1  1  1]"  x_out=[0.6 0.68 0.68 0.76 0.76 0.84 0.84 0.92 0.92 1]  y_out="[-1 -1  1  1 -1 -1 -1 -1 -1 -1]"
  edge_detect1 : casper_library_misc/edge_detect  edge=Rising  polarity=Active High  x_in=[0 0.08 0.08 0.16 0.16 0.24 0.24 0.32 0.32 0.4]  y_in="[-1 -1  1  1  1  1  1  1  1  1]"  x_out=[0.6 0.68 0.68 0.76 0.76 0.84 0.84 0.92 0.92 1]  y_out="[-1 -1  1  1 -1 -1 -1 -1 -1 -1]"
  pipeline1 : Subsystem  AncestorBlock=casper_library_delays/pipeline  mask(pipeline){latency=2}
      mask help:
      | An explicitly laid-out delay line to avoid mapping to SRL16s
      | for use in pipelining to help achieve timing closure.
      mask init:
      | pipeline_init(gcb,'latency',latency);
      settings: AttributesFormatString=Latency = %<latency>
      mask Display:
      | port_label('input', 1, 'd');
      | port_label('output', 1, 'q');
      | disp(['Z^-', num2str(latency)]);
  pipeline2 : Subsystem  AncestorBlock=casper_library_delays/pipeline  mask(pipeline){latency=2}
      mask help:
      | An explicitly laid-out delay line to avoid mapping to SRL16s
      | for use in pipelining to help achieve timing closure.
      mask init:
      | pipeline_init(gcb,'latency',latency);
      settings: AttributesFormatString=Latency = %<latency>
      mask Display:
      | port_label('input', 1, 'd');
      | port_label('output', 1, 'q');
      | disp(['Z^-', num2str(latency)]);
  pipeline53 : Subsystem  AncestorBlock=casper_library_delays/pipeline  mask(pipeline){latency=2}
      mask help:
      | An explicitly laid-out delay line to avoid mapping to SRL16s
      | for use in pipelining to help achieve timing closure.
      mask init:
      | pipeline_init(gcb,'latency',latency);
      settings: AttributesFormatString=Latency = %<latency>
      mask Display:
      | port_label('input', 1, 'd');
      | port_label('output', 1, 'q');
      | disp(['Z^-', num2str(latency)]);
  pipeline54 : Subsystem  AncestorBlock=casper_library_delays/pipeline  mask(pipeline){latency=2}
      mask help:
      | An explicitly laid-out delay line to avoid mapping to SRL16s
      | for use in pipelining to help achieve timing closure.
      mask init:
      | pipeline_init(gcb,'latency',latency);
      settings: AttributesFormatString=Latency = %<latency>
      mask Display:
      | port_label('input', 1, 'd');
      | port_label('output', 1, 'q');
      | disp(['Z^-', num2str(latency)]);
  pipeline55 : Subsystem  AncestorBlock=casper_library_delays/pipeline  mask(pipeline){latency=2}
      mask help:
      | An explicitly laid-out delay line to avoid mapping to SRL16s
      | for use in pipelining to help achieve timing closure.
      mask init:
      | pipeline_init(gcb,'latency',latency);
      settings: AttributesFormatString=Latency = %<latency>
      mask Display:
      | port_label('input', 1, 'd');
      | port_label('output', 1, 'q');
      | disp(['Z^-', num2str(latency)]);
  pipeline7 : Subsystem  AncestorBlock=casper_library_delays/pipeline  mask(pipeline){latency=2}
      mask help:
      | An explicitly laid-out delay line to avoid mapping to SRL16s
      | for use in pipelining to help achieve timing closure.
      mask init:
      | pipeline_init(gcb,'latency',latency);
      settings: AttributesFormatString=Latency = %<latency>
      mask Display:
      | port_label('input', 1, 'd');
      | port_label('output', 1, 'q');
      | disp(['Z^-', num2str(latency)]);
  Out1 : Outport
  Out2 : Outport  Port=2
  wires:
  pipeline55/1(q) -> Out1/1
  pipeline7/1(q) -> Out2/1
  Counter1/1 -> pipeline7/1(d)
  in1/1 -> pipeline2/1(d)
  pipeline2/1(q) -> edge_detect1/1
  edge_detect1/1 -> Counter1/2
  pipeline1/1(q) -> Counter1/1
  edge_detect/1 -> Counter/2
  rst/1 -> pipeline53/1(d), pipeline1/1(d)
  pipeline53/1(q) -> Counter/1
  pipeline54/1(q) -> edge_detect/1
  Counter/1 -> pipeline55/1(d)
  in0/1 -> pipeline54/1(d)
